simulink model "induction_motor_basics"  (R2021a)
settings: Solver=VariableStepAuto  StartTime=0.0  StopTime=2.0  RelTol=1e-3
libraries: spsAsynchronousMachineSIUnitsLib x1, spsThreePhaseSourceLib x1, spspowerguiLib x1
settings Model: Creator=Prakhar  LastModifiedBy=Prakhar

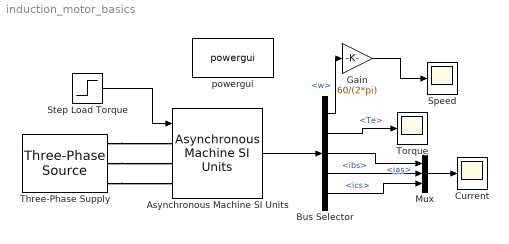
== system induction_motor_basics ==
  Asynchronous Machine SI Units : spsAsynchronousMachineSIUnitsLib/Asynchronous Machine SI Units  RotorType=Squirrel-cage  PresetModel=No  MechanicalLoad=Torque Tm  ShowDetailedParameters=on  ReferenceFrame=Rotor  Units=SI  MeasurementBus=on  NominalParameters=[5.5e3 400 50]  VoltageRatio=1  Stator=[0.5 0.00382]  Rotor=[0.3 0.002546]  Cage1=[0.4155 0.002066]  Cage2=[0.4168 0.0003495]  Lm=0.09549  Mechanical=[0.05 0.001 2]  PolePairs=2  InitialConditions=[0 0 0 0 0 0 0 0]  SimulateSaturation=off  Saturation=[14.03593122, 27.81365428, 53.79336849, 72.68890987, 97.98006896, 148.6815601, 215.7428561, 302.9841135, 428.7778367 ; 230, 322, 414, 460, 506, 552, 598, 644, 690]  LoadFlowParameters=1492000  TsPowergui=0  TsBlock=-1  IterativeModel=Trapezoidal non iterative  IterativeDiscreteModel=Trapezoidal non iterative  Pmec=1.492e+006
  Bus Selector : BusSelector  OutputSignals=w,Te,ias,ibs,ics
  Current : Scope
  Gain : Gain  Gain=60/(2*pi)
  Mux : Mux  Inputs=3
  Speed : Scope
  Step Load Torque : Step  After=20  SampleTime=0
  Three-Phase Supply : spsThreePhaseSourceLib/Three-Phase Source  InternalConnection=Yg  VoltagePhases=off  Voltage=400  PhaseAngle=0  Voltage_phases=[25e3 25e3 25e3]/sqrt(3)  PhaseAngles_phases=[0 -120 +120]  Frequency=50  NonIdealSource=off  SpecifyImpedance=off  Resistance=0.8929  Inductance=16.58e-3  ShortCircuitLevel=100e6  BaseVoltage=25e3  XRratio=7  BusType=swing  Pref=10e3  Qref=0  Prefabc=[10e3, 10e3, 10e3]  Qrefabc=[0, 0, 0]  Qmin=-inf  Qmax=inf
  Torque : Scope
  powergui : spspowerguiLib/powergui  Priority=1  SimulationMode=Continuous  SampleTime=50e-6  frequency=60  Iterations=50  frequencyindice=50  Pbase=100e6  ErrMax=1e-4  UnitsV=kV  UnitsW=MW  buscounter=0  FunctionMessages=off  echomessages=off  EnableUseOfTLC=off  CurrentSourceSwitches=off  DisableSnubberDevices=off  DisableRonSwitches=off  DisableVfSwitches=off  DisplayEquations=off  AutomaticDiscreteSolvers=off  SolverType=Tustin/Backward Euler (TBE)  Interpol=off  ExternalGateDelay=off  methode=off  Ts=100  x0status=blocks  SPID=on  SwTol=0  HookPort=off  NonlinearTolerance=1e-4  nMaxIteration=100  ContinueOnMaxIteration=off  RestoreLinks=warning  ResistiveCurrentMeasurement=off  Frange=[0:2:500]  Ylog=off  Xlog=on  ShowGrid=off  save=off  variable=ZData  structure=0  ZoomFFT=off  StartTime=0.0  cycles=1  DisplayStyle=1  fundamental=60  FreqAxis=off  MaxFrequency=1000  frequencyindicesteady=1  RmsSteady=1  display=off
  wires:
  Bus Selector/3 -> Mux/1  "<ias>"
  Bus Selector/4 -> Mux/2  "<ibs>"
  Bus Selector/5 -> Mux/3  "<ics>"
  Bus Selector/2 -> Torque/1  "<Te>"
  Mux/1 -> Current/1
  Bus Selector/1 -> Gain/1  "<w>"
  Step Load Torque/1 -> Asynchronous Machine SI Units/1
  Asynchronous Machine SI Units/1 -> Bus Selector/1
  Gain/1 -> Speed/1
  connections:
  Three-Phase Supply/RConn1 -- Asynchronous Machine SI Units/LConn1
  Three-Phase Supply/RConn2 -- Asynchronous Machine SI Units/LConn2
  Three-Phase Supply/RConn3 -- Asynchronous Machine SI Units/LConn3
